simulink model "EV_Truck_Model"  (R2022b)
settings: Solver=FixedStepAuto  StartTime=0  StopTime=26553  FixedStep=0.1  RelTol=1e-3
model workspace (MAT data in the model file):
  ADAS_MaxAccel = 2
  ADAS_MaxDecel = 2.5
  Adas_on_off = 0
  Batt_cap_ah : Simulink.Parameter (value not decoded)
  Batt_rist_r0 : Simulink.Parameter (value not decoded)
  Batt_soc_s0 : Simulink.Parameter (value not decoded)
  Batt_volt_v0 : Simulink.Parameter (value not decoded)
  Motor_eff_100 : Simulink.Parameter (value not decoded)
  Motor_eff_190 : Simulink.Parameter (value not decoded)
  Motor_eff_95 : Simulink.Parameter (value not decoded)
  Motor_rpm_100 : Simulink.Parameter (value not decoded)
  Motor_rpm_190 : Simulink.Parameter (value not decoded)
  Motor_rpm_95 : Simulink.Parameter (value not decoded)
  Motor_torque_pos_100 : Simulink.Parameter (value not decoded)
  Motor_torque_pos_190 : Simulink.Parameter (value not decoded)
  Motor_torque_pos_95 : Simulink.Parameter (value not decoded)
  Motor_trq_190 : Simulink.Parameter (value not decoded)
  Motor_trq_95 : Simulink.Parameter (value not decoded)
  Sim_step = 0.1
  Test_DriveCycle = 0
  Trans_ratio = 6.142
  Veh_cog_fx = 1.69543
  Veh_cog_h = 0.605887
  Veh_cog_rx = 2.11956
  Veh_diff = 6.7
  Veh_whl_crr = 0.01
  Veh_whl_k = 180000
  Veh_whl_radius = 0.35
symbols that are objects in the model workspace (value not decoded): Motor_eff_100, Motor_eff_190, Motor_eff_95, Motor_rpm_100, Motor_rpm_190, Motor_rpm_95, Motor_torque_pos_100, Motor_torque_pos_190, Motor_torque_pos_95, Motor_trq_190, Motor_trq_95
undefined symbols (not defined in the file): Batt_soc_init, canChannel, Elec_aux_sw, Elec_rgn_sw, Power_option, speed, time, Veh_mass
libraries: batteryecm_lib x170, simulink x14, canmsglib x9, canlib x7, autolibshared x5, nesl_utility x4, fl_lib x3, drivingvehiclecontroller x3, hdlsllib x3, sim3dlib x1, sim3dautolib x1, vrlib x1
(part 6 of 11)

== system EV_Truck_Model/Accumulator System/Battery Pack/Simscape HV Battery/Battery Semi-Pack 1 ==
  Battery 7s6p1 : Subsystem
      settings: PortSchema="{\"entries\":[{\"content\":{\"sides\":[{\"content\":{\"connectorIds\":[]},\"type\":\"ConnectorPlacement.EquallySpacedRectSide\",\"uuid\":\"a0694fe7-d780-4483-a41f-a7ed21683973\"},{\"content\":{\"connectorIds\":[],\"side\":\"RIGHT\"},\"type\":\"ConnectorPlacement.EquallySpacedRectSide\",\"uuid\":\"39469ca5-beea-4553-8147-277bd4be0bbc\"},{\"content\":{\"connectorIds\":[\"LConn1\"],\"side\":\"TOP\"},\"type\":\"ConnectorPlacement.EquallySpacedRectSide\",\"uuid\":\"ededc17a-74df-4b2c-b94f-9a58df69fee7\"},{\"content\":{\"connectorIds\":[\"RConn1\"],\"side\":\"BOTTOM\"},\"type\":\"ConnectorPlacement.EquallySpacedRectSide\",\"uuid\":\"b7141beb-a775-4bdc-a667-5b3929cade8e\"}]},\"type\":\"ConnectorPlacement.EquallySpacedConnector\",\"uuid\":\"2df81f02-ea4e-4946-bfe6-2aa0de3e9d2a\"}],\"packageUris\":[\"http://schema.mathworks.com/mf0/Connector/R2020b\"],\"version\":\"1.0\"}"
  Battery 7s6p2 : Subsystem
      settings: PortSchema="{\"entries\":[{\"content\":{\"sides\":[{\"content\":{\"connectorIds\":[]},\"type\":\"ConnectorPlacement.EquallySpacedRectSide\",\"uuid\":\"a0694fe7-d780-4483-a41f-a7ed21683973\"},{\"content\":{\"connectorIds\":[],\"side\":\"RIGHT\"},\"type\":\"ConnectorPlacement.EquallySpacedRectSide\",\"uuid\":\"39469ca5-beea-4553-8147-277bd4be0bbc\"},{\"content\":{\"connectorIds\":[\"LConn1\"],\"side\":\"TOP\"},\"type\":\"ConnectorPlacement.EquallySpacedRectSide\",\"uuid\":\"ededc17a-74df-4b2c-b94f-9a58df69fee7\"},{\"content\":{\"connectorIds\":[\"RConn1\"],\"side\":\"BOTTOM\"},\"type\":\"ConnectorPlacement.EquallySpacedRectSide\",\"uuid\":\"b7141beb-a775-4bdc-a667-5b3929cade8e\"}]},\"type\":\"ConnectorPlacement.EquallySpacedConnector\",\"uuid\":\"2df81f02-ea4e-4946-bfe6-2aa0de3e9d2a\"}],\"packageUris\":[\"http://schema.mathworks.com/mf0/Connector/R2020b\"],\"version\":\"1.0\"}"
  Battery 7s6p3 : Subsystem
      settings: PortSchema="{\"entries\":[{\"content\":{\"sides\":[{\"content\":{\"connectorIds\":[]},\"type\":\"ConnectorPlacement.EquallySpacedRectSide\",\"uuid\":\"a0694fe7-d780-4483-a41f-a7ed21683973\"},{\"content\":{\"connectorIds\":[],\"side\":\"RIGHT\"},\"type\":\"ConnectorPlacement.EquallySpacedRectSide\",\"uuid\":\"39469ca5-beea-4553-8147-277bd4be0bbc\"},{\"content\":{\"connectorIds\":[\"LConn1\"],\"side\":\"TOP\"},\"type\":\"ConnectorPlacement.EquallySpacedRectSide\",\"uuid\":\"ededc17a-74df-4b2c-b94f-9a58df69fee7\"},{\"content\":{\"connectorIds\":[\"RConn1\"],\"side\":\"BOTTOM\"},\"type\":\"ConnectorPlacement.EquallySpacedRectSide\",\"uuid\":\"b7141beb-a775-4bdc-a667-5b3929cade8e\"}]},\"type\":\"ConnectorPlacement.EquallySpacedConnector\",\"uuid\":\"2df81f02-ea4e-4946-bfe6-2aa0de3e9d2a\"}],\"packageUris\":[\"http://schema.mathworks.com/mf0/Connector/R2020b\"],\"version\":\"1.0\"}"
  Battery 7s6p4 : Subsystem
      settings: PortSchema="{\"entries\":[{\"content\":{\"sides\":[{\"content\":{\"connectorIds\":[]},\"type\":\"ConnectorPlacement.EquallySpacedRectSide\",\"uuid\":\"a0694fe7-d780-4483-a41f-a7ed21683973\"},{\"content\":{\"connectorIds\":[],\"side\":\"RIGHT\"},\"type\":\"ConnectorPlacement.EquallySpacedRectSide\",\"uuid\":\"39469ca5-beea-4553-8147-277bd4be0bbc\"},{\"content\":{\"connectorIds\":[\"LConn1\"],\"side\":\"TOP\"},\"type\":\"ConnectorPlacement.EquallySpacedRectSide\",\"uuid\":\"ededc17a-74df-4b2c-b94f-9a58df69fee7\"},{\"content\":{\"connectorIds\":[\"RConn1\"],\"side\":\"BOTTOM\"},\"type\":\"ConnectorPlacement.EquallySpacedRectSide\",\"uuid\":\"b7141beb-a775-4bdc-a667-5b3929cade8e\"}]},\"type\":\"ConnectorPlacement.EquallySpacedConnector\",\"uuid\":\"2df81f02-ea4e-4946-bfe6-2aa0de3e9d2a\"}],\"packageUris\":[\"http://schema.mathworks.com/mf0/Connector/R2020b\"],\"version\":\"1.0\"}"
  Battery 7s6p5 : Subsystem
      settings: PortSchema="{\"entries\":[{\"content\":{\"sides\":[{\"content\":{\"connectorIds\":[]},\"type\":\"ConnectorPlacement.EquallySpacedRectSide\",\"uuid\":\"a0694fe7-d780-4483-a41f-a7ed21683973\"},{\"content\":{\"connectorIds\":[],\"side\":\"RIGHT\"},\"type\":\"ConnectorPlacement.EquallySpacedRectSide\",\"uuid\":\"39469ca5-beea-4553-8147-277bd4be0bbc\"},{\"content\":{\"connectorIds\":[\"LConn1\"],\"side\":\"TOP\"},\"type\":\"ConnectorPlacement.EquallySpacedRectSide\",\"uuid\":\"ededc17a-74df-4b2c-b94f-9a58df69fee7\"},{\"content\":{\"connectorIds\":[\"RConn1\"],\"side\":\"BOTTOM\"},\"type\":\"ConnectorPlacement.EquallySpacedRectSide\",\"uuid\":\"b7141beb-a775-4bdc-a667-5b3929cade8e\"}]},\"type\":\"ConnectorPlacement.EquallySpacedConnector\",\"uuid\":\"2df81f02-ea4e-4946-bfe6-2aa0de3e9d2a\"}],\"packageUris\":[\"http://schema.mathworks.com/mf0/Connector/R2020b\"],\"version\":\"1.0\"}"
  Battery 7s6p6 : Subsystem
      settings: PortSchema="{\"entries\":[{\"content\":{\"sides\":[{\"content\":{\"connectorIds\":[]},\"type\":\"ConnectorPlacement.EquallySpacedRectSide\",\"uuid\":\"a0694fe7-d780-4483-a41f-a7ed21683973\"},{\"content\":{\"connectorIds\":[],\"side\":\"RIGHT\"},\"type\":\"ConnectorPlacement.EquallySpacedRectSide\",\"uuid\":\"39469ca5-beea-4553-8147-277bd4be0bbc\"},{\"content\":{\"connectorIds\":[\"LConn1\"],\"side\":\"TOP\"},\"type\":\"ConnectorPlacement.EquallySpacedRectSide\",\"uuid\":\"ededc17a-74df-4b2c-b94f-9a58df69fee7\"},{\"content\":{\"connectorIds\":[\"RConn1\"],\"side\":\"BOTTOM\"},\"type\":\"ConnectorPlacement.EquallySpacedRectSide\",\"uuid\":\"b7141beb-a775-4bdc-a667-5b3929cade8e\"}]},\"type\":\"ConnectorPlacement.EquallySpacedConnector\",\"uuid\":\"2df81f02-ea4e-4946-bfe6-2aa0de3e9d2a\"}],\"packageUris\":[\"http://schema.mathworks.com/mf0/Connector/R2020b\"],\"version\":\"1.0\"}"
  High : PMIOPort  Side=Left
  Low : PMIOPort  Port=2  Side=Right
  connections:
  Battery 7s6p2/LConn1 -- Battery 7s6p1/RConn1
  High/RConn1 -- Battery 7s6p1/LConn1
  Battery 7s6p6/RConn1 -- Low/RConn1
  Battery 7s6p3/LConn1 -- Battery 7s6p2/RConn1
  Battery 7s6p4/LConn1 -- Battery 7s6p3/RConn1
  Battery 7s6p5/RConn1 -- Battery 7s6p6/LConn1
  Battery 7s6p5/LConn1 -- Battery 7s6p4/RConn1

== system EV_Truck_Model/Accumulator System/Battery Pack/Simscape HV Battery/Battery Semi-Pack 2 ==
  Battery 7s6p1 : Subsystem
      settings: PortSchema="{\"entries\":[{\"content\":{\"sides\":[{\"content\":{\"connectorIds\":[]},\"type\":\"ConnectorPlacement.EquallySpacedRectSide\",\"uuid\":\"a0694fe7-d780-4483-a41f-a7ed21683973\"},{\"content\":{\"connectorIds\":[],\"side\":\"RIGHT\"},\"type\":\"ConnectorPlacement.EquallySpacedRectSide\",\"uuid\":\"39469ca5-beea-4553-8147-277bd4be0bbc\"},{\"content\":{\"connectorIds\":[\"LConn1\"],\"side\":\"TOP\"},\"type\":\"ConnectorPlacement.EquallySpacedRectSide\",\"uuid\":\"ededc17a-74df-4b2c-b94f-9a58df69fee7\"},{\"content\":{\"connectorIds\":[\"RConn1\"],\"side\":\"BOTTOM\"},\"type\":\"ConnectorPlacement.EquallySpacedRectSide\",\"uuid\":\"b7141beb-a775-4bdc-a667-5b3929cade8e\"}]},\"type\":\"ConnectorPlacement.EquallySpacedConnector\",\"uuid\":\"2df81f02-ea4e-4946-bfe6-2aa0de3e9d2a\"}],\"packageUris\":[\"http://schema.mathworks.com/mf0/Connector/R2020b\"],\"version\":\"1.0\"}"
  Battery 7s6p2 : Subsystem
      settings: PortSchema="{\"entries\":[{\"content\":{\"sides\":[{\"content\":{\"connectorIds\":[]},\"type\":\"ConnectorPlacement.EquallySpacedRectSide\",\"uuid\":\"a0694fe7-d780-4483-a41f-a7ed21683973\"},{\"content\":{\"connectorIds\":[],\"side\":\"RIGHT\"},\"type\":\"ConnectorPlacement.EquallySpacedRectSide\",\"uuid\":\"39469ca5-beea-4553-8147-277bd4be0bbc\"},{\"content\":{\"connectorIds\":[\"LConn1\"],\"side\":\"TOP\"},\"type\":\"ConnectorPlacement.EquallySpacedRectSide\",\"uuid\":\"ededc17a-74df-4b2c-b94f-9a58df69fee7\"},{\"content\":{\"connectorIds\":[\"RConn1\"],\"side\":\"BOTTOM\"},\"type\":\"ConnectorPlacement.EquallySpacedRectSide\",\"uuid\":\"b7141beb-a775-4bdc-a667-5b3929cade8e\"}]},\"type\":\"ConnectorPlacement.EquallySpacedConnector\",\"uuid\":\"2df81f02-ea4e-4946-bfe6-2aa0de3e9d2a\"}],\"packageUris\":[\"http://schema.mathworks.com/mf0/Connector/R2020b\"],\"version\":\"1.0\"}"
  Battery 7s6p3 : Subsystem
      settings: PortSchema="{\"entries\":[{\"content\":{\"sides\":[{\"content\":{\"connectorIds\":[]},\"type\":\"ConnectorPlacement.EquallySpacedRectSide\",\"uuid\":\"a0694fe7-d780-4483-a41f-a7ed21683973\"},{\"content\":{\"connectorIds\":[],\"side\":\"RIGHT\"},\"type\":\"ConnectorPlacement.EquallySpacedRectSide\",\"uuid\":\"39469ca5-beea-4553-8147-277bd4be0bbc\"},{\"content\":{\"connectorIds\":[\"LConn1\"],\"side\":\"TOP\"},\"type\":\"ConnectorPlacement.EquallySpacedRectSide\",\"uuid\":\"ededc17a-74df-4b2c-b94f-9a58df69fee7\"},{\"content\":{\"connectorIds\":[\"RConn1\"],\"side\":\"BOTTOM\"},\"type\":\"ConnectorPlacement.EquallySpacedRectSide\",\"uuid\":\"b7141beb-a775-4bdc-a667-5b3929cade8e\"}]},\"type\":\"ConnectorPlacement.EquallySpacedConnector\",\"uuid\":\"2df81f02-ea4e-4946-bfe6-2aa0de3e9d2a\"}],\"packageUris\":[\"http://schema.mathworks.com/mf0/Connector/R2020b\"],\"version\":\"1.0\"}"
  Battery 7s6p4 : Subsystem
      settings: PortSchema="{\"entries\":[{\"content\":{\"sides\":[{\"content\":{\"connectorIds\":[]},\"type\":\"ConnectorPlacement.EquallySpacedRectSide\",\"uuid\":\"a0694fe7-d780-4483-a41f-a7ed21683973\"},{\"content\":{\"connectorIds\":[],\"side\":\"RIGHT\"},\"type\":\"ConnectorPlacement.EquallySpacedRectSide\",\"uuid\":\"39469ca5-beea-4553-8147-277bd4be0bbc\"},{\"content\":{\"connectorIds\":[\"LConn1\"],\"side\":\"TOP\"},\"type\":\"ConnectorPlacement.EquallySpacedRectSide\",\"uuid\":\"ededc17a-74df-4b2c-b94f-9a58df69fee7\"},{\"content\":{\"connectorIds\":[\"RConn1\"],\"side\":\"BOTTOM\"},\"type\":\"ConnectorPlacement.EquallySpacedRectSide\",\"uuid\":\"b7141beb-a775-4bdc-a667-5b3929cade8e\"}]},\"type\":\"ConnectorPlacement.EquallySpacedConnector\",\"uuid\":\"2df81f02-ea4e-4946-bfe6-2aa0de3e9d2a\"}],\"packageUris\":[\"http://schema.mathworks.com/mf0/Connector/R2020b\"],\"version\":\"1.0\"}"
  Battery 7s6p5 : Subsystem
      settings: PortSchema="{\"entries\":[{\"content\":{\"sides\":[{\"content\":{\"connectorIds\":[]},\"type\":\"ConnectorPlacement.EquallySpacedRectSide\",\"uuid\":\"a0694fe7-d780-4483-a41f-a7ed21683973\"},{\"content\":{\"connectorIds\":[],\"side\":\"RIGHT\"},\"type\":\"ConnectorPlacement.EquallySpacedRectSide\",\"uuid\":\"39469ca5-beea-4553-8147-277bd4be0bbc\"},{\"content\":{\"connectorIds\":[\"LConn1\"],\"side\":\"TOP\"},\"type\":\"ConnectorPlacement.EquallySpacedRectSide\",\"uuid\":\"ededc17a-74df-4b2c-b94f-9a58df69fee7\"},{\"content\":{\"connectorIds\":[\"RConn1\"],\"side\":\"BOTTOM\"},\"type\":\"ConnectorPlacement.EquallySpacedRectSide\",\"uuid\":\"b7141beb-a775-4bdc-a667-5b3929cade8e\"}]},\"type\":\"ConnectorPlacement.EquallySpacedConnector\",\"uuid\":\"2df81f02-ea4e-4946-bfe6-2aa0de3e9d2a\"}],\"packageUris\":[\"http://schema.mathworks.com/mf0/Connector/R2020b\"],\"version\":\"1.0\"}"
  Battery 7s6p6 : Subsystem
      settings: PortSchema="{\"entries\":[{\"content\":{\"sides\":[{\"content\":{\"connectorIds\":[]},\"type\":\"ConnectorPlacement.EquallySpacedRectSide\",\"uuid\":\"a0694fe7-d780-4483-a41f-a7ed21683973\"},{\"content\":{\"connectorIds\":[],\"side\":\"RIGHT\"},\"type\":\"ConnectorPlacement.EquallySpacedRectSide\",\"uuid\":\"39469ca5-beea-4553-8147-277bd4be0bbc\"},{\"content\":{\"connectorIds\":[\"LConn1\"],\"side\":\"TOP\"},\"type\":\"ConnectorPlacement.EquallySpacedRectSide\",\"uuid\":\"ededc17a-74df-4b2c-b94f-9a58df69fee7\"},{\"content\":{\"connectorIds\":[\"RConn1\"],\"side\":\"BOTTOM\"},\"type\":\"ConnectorPlacement.EquallySpacedRectSide\",\"uuid\":\"b7141beb-a775-4bdc-a667-5b3929cade8e\"}]},\"type\":\"ConnectorPlacement.EquallySpacedConnector\",\"uuid\":\"2df81f02-ea4e-4946-bfe6-2aa0de3e9d2a\"}],\"packageUris\":[\"http://schema.mathworks.com/mf0/Connector/R2020b\"],\"version\":\"1.0\"}"
  High : PMIOPort  Side=Left
  Low : PMIOPort  Port=2  Side=Right
  connections:
  Battery 7s6p2/LConn1 -- Battery 7s6p1/RConn1
  High/RConn1 -- Battery 7s6p1/LConn1
  Battery 7s6p6/RConn1 -- Low/RConn1
  Battery 7s6p3/LConn1 -- Battery 7s6p2/RConn1
  Battery 7s6p4/LConn1 -- Battery 7s6p3/RConn1
  Battery 7s6p5/RConn1 -- Battery 7s6p6/LConn1
  Battery 7s6p5/LConn1 -- Battery 7s6p4/RConn1

== system EV_Truck_Model/Accumulator System/Battery Pack/Simscape HV Battery/Battery Semi-Pack 3 ==
  Battery 7s6p1 : Subsystem
      settings: PortSchema="{\"entries\":[{\"content\":{\"sides\":[{\"content\":{\"connectorIds\":[]},\"type\":\"ConnectorPlacement.EquallySpacedRectSide\",\"uuid\":\"a0694fe7-d780-4483-a41f-a7ed21683973\"},{\"content\":{\"connectorIds\":[],\"side\":\"RIGHT\"},\"type\":\"ConnectorPlacement.EquallySpacedRectSide\",\"uuid\":\"39469ca5-beea-4553-8147-277bd4be0bbc\"},{\"content\":{\"connectorIds\":[\"LConn1\"],\"side\":\"TOP\"},\"type\":\"ConnectorPlacement.EquallySpacedRectSide\",\"uuid\":\"ededc17a-74df-4b2c-b94f-9a58df69fee7\"},{\"content\":{\"connectorIds\":[\"RConn1\"],\"side\":\"BOTTOM\"},\"type\":\"ConnectorPlacement.EquallySpacedRectSide\",\"uuid\":\"b7141beb-a775-4bdc-a667-5b3929cade8e\"}]},\"type\":\"ConnectorPlacement.EquallySpacedConnector\",\"uuid\":\"2df81f02-ea4e-4946-bfe6-2aa0de3e9d2a\"}],\"packageUris\":[\"http://schema.mathworks.com/mf0/Connector/R2020b\"],\"version\":\"1.0\"}"
  Battery 7s6p2 : Subsystem
      settings: PortSchema="{\"entries\":[{\"content\":{\"sides\":[{\"content\":{\"connectorIds\":[]},\"type\":\"ConnectorPlacement.EquallySpacedRectSide\",\"uuid\":\"a0694fe7-d780-4483-a41f-a7ed21683973\"},{\"content\":{\"connectorIds\":[],\"side\":\"RIGHT\"},\"type\":\"ConnectorPlacement.EquallySpacedRectSide\",\"uuid\":\"39469ca5-beea-4553-8147-277bd4be0bbc\"},{\"content\":{\"connectorIds\":[\"LConn1\"],\"side\":\"TOP\"},\"type\":\"ConnectorPlacement.EquallySpacedRectSide\",\"uuid\":\"ededc17a-74df-4b2c-b94f-9a58df69fee7\"},{\"content\":{\"connectorIds\":[\"RConn1\"],\"side\":\"BOTTOM\"},\"type\":\"ConnectorPlacement.EquallySpacedRectSide\",\"uuid\":\"b7141beb-a775-4bdc-a667-5b3929cade8e\"}]},\"type\":\"ConnectorPlacement.EquallySpacedConnector\",\"uuid\":\"2df81f02-ea4e-4946-bfe6-2aa0de3e9d2a\"}],\"packageUris\":[\"http://schema.mathworks.com/mf0/Connector/R2020b\"],\"version\":\"1.0\"}"
  Battery 7s6p3 : Subsystem
      settings: PortSchema="{\"entries\":[{\"content\":{\"sides\":[{\"content\":{\"connectorIds\":[]},\"type\":\"ConnectorPlacement.EquallySpacedRectSide\",\"uuid\":\"a0694fe7-d780-4483-a41f-a7ed21683973\"},{\"content\":{\"connectorIds\":[],\"side\":\"RIGHT\"},\"type\":\"ConnectorPlacement.EquallySpacedRectSide\",\"uuid\":\"39469ca5-beea-4553-8147-277bd4be0bbc\"},{\"content\":{\"connectorIds\":[\"LConn1\"],\"side\":\"TOP\"},\"type\":\"ConnectorPlacement.EquallySpacedRectSide\",\"uuid\":\"ededc17a-74df-4b2c-b94f-9a58df69fee7\"},{\"content\":{\"connectorIds\":[\"RConn1\"],\"side\":\"BOTTOM\"},\"type\":\"ConnectorPlacement.EquallySpacedRectSide\",\"uuid\":\"b7141beb-a775-4bdc-a667-5b3929cade8e\"}]},\"type\":\"ConnectorPlacement.EquallySpacedConnector\",\"uuid\":\"2df81f02-ea4e-4946-bfe6-2aa0de3e9d2a\"}],\"packageUris\":[\"http://schema.mathworks.com/mf0/Connector/R2020b\"],\"version\":\"1.0\"}"
  Battery 7s6p4 : Subsystem
      settings: PortSchema="{\"entries\":[{\"content\":{\"sides\":[{\"content\":{\"connectorIds\":[]},\"type\":\"ConnectorPlacement.EquallySpacedRectSide\",\"uuid\":\"a0694fe7-d780-4483-a41f-a7ed21683973\"},{\"content\":{\"connectorIds\":[],\"side\":\"RIGHT\"},\"type\":\"ConnectorPlacement.EquallySpacedRectSide\",\"uuid\":\"39469ca5-beea-4553-8147-277bd4be0bbc\"},{\"content\":{\"connectorIds\":[\"LConn1\"],\"side\":\"TOP\"},\"type\":\"ConnectorPlacement.EquallySpacedRectSide\",\"uuid\":\"ededc17a-74df-4b2c-b94f-9a58df69fee7\"},{\"content\":{\"connectorIds\":[\"RConn1\"],\"side\":\"BOTTOM\"},\"type\":\"ConnectorPlacement.EquallySpacedRectSide\",\"uuid\":\"b7141beb-a775-4bdc-a667-5b3929cade8e\"}]},\"type\":\"ConnectorPlacement.EquallySpacedConnector\",\"uuid\":\"2df81f02-ea4e-4946-bfe6-2aa0de3e9d2a\"}],\"packageUris\":[\"http://schema.mathworks.com/mf0/Connector/R2020b\"],\"version\":\"1.0\"}"
  Battery 7s6p5 : Subsystem
      settings: PortSchema="{\"entries\":[{\"content\":{\"sides\":[{\"content\":{\"connectorIds\":[]},\"type\":\"ConnectorPlacement.EquallySpacedRectSide\",\"uuid\":\"a0694fe7-d780-4483-a41f-a7ed21683973\"},{\"content\":{\"connectorIds\":[],\"side\":\"RIGHT\"},\"type\":\"ConnectorPlacement.EquallySpacedRectSide\",\"uuid\":\"39469ca5-beea-4553-8147-277bd4be0bbc\"},{\"content\":{\"connectorIds\":[\"LConn1\"],\"side\":\"TOP\"},\"type\":\"ConnectorPlacement.EquallySpacedRectSide\",\"uuid\":\"ededc17a-74df-4b2c-b94f-9a58df69fee7\"},{\"content\":{\"connectorIds\":[\"RConn1\"],\"side\":\"BOTTOM\"},\"type\":\"ConnectorPlacement.EquallySpacedRectSide\",\"uuid\":\"b7141beb-a775-4bdc-a667-5b3929cade8e\"}]},\"type\":\"ConnectorPlacement.EquallySpacedConnector\",\"uuid\":\"2df81f02-ea4e-4946-bfe6-2aa0de3e9d2a\"}],\"packageUris\":[\"http://schema.mathworks.com/mf0/Connector/R2020b\"],\"version\":\"1.0\"}"
  Battery 7s6p6 : Subsystem
      settings: PortSchema="{\"entries\":[{\"content\":{\"sides\":[{\"content\":{\"connectorIds\":[]},\"type\":\"ConnectorPlacement.EquallySpacedRectSide\",\"uuid\":\"a0694fe7-d780-4483-a41f-a7ed21683973\"},{\"content\":{\"connectorIds\":[],\"side\":\"RIGHT\"},\"type\":\"ConnectorPlacement.EquallySpacedRectSide\",\"uuid\":\"39469ca5-beea-4553-8147-277bd4be0bbc\"},{\"content\":{\"connectorIds\":[\"LConn1\"],\"side\":\"TOP\"},\"type\":\"ConnectorPlacement.EquallySpacedRectSide\",\"uuid\":\"ededc17a-74df-4b2c-b94f-9a58df69fee7\"},{\"content\":{\"connectorIds\":[\"RConn1\"],\"side\":\"BOTTOM\"},\"type\":\"ConnectorPlacement.EquallySpacedRectSide\",\"uuid\":\"b7141beb-a775-4bdc-a667-5b3929cade8e\"}]},\"type\":\"ConnectorPlacement.EquallySpacedConnector\",\"uuid\":\"2df81f02-ea4e-4946-bfe6-2aa0de3e9d2a\"}],\"packageUris\":[\"http://schema.mathworks.com/mf0/Connector/R2020b\"],\"version\":\"1.0\"}"
  High : PMIOPort  Side=Left
  Low : PMIOPort  Port=2  Side=Right
  connections:
  Battery 7s6p2/LConn1 -- Battery 7s6p1/RConn1
  High/RConn1 -- Battery 7s6p1/LConn1
  Battery 7s6p6/RConn1 -- Low/RConn1
  Battery 7s6p3/LConn1 -- Battery 7s6p2/RConn1
  Battery 7s6p4/LConn1 -- Battery 7s6p3/RConn1
  Battery 7s6p5/RConn1 -- Battery 7s6p6/LConn1
  Battery 7s6p5/LConn1 -- Battery 7s6p4/RConn1

== system EV_Truck_Model/Accumulator System/Battery Pack/Simscape HV Battery/Battery Semi-Pack 4 ==
  Battery 7s6p1 : Subsystem
      settings: PortSchema="{\"entries\":[{\"content\":{\"sides\":[{\"content\":{\"connectorIds\":[]},\"type\":\"ConnectorPlacement.EquallySpacedRectSide\",\"uuid\":\"a0694fe7-d780-4483-a41f-a7ed21683973\"},{\"content\":{\"connectorIds\":[],\"side\":\"RIGHT\"},\"type\":\"ConnectorPlacement.EquallySpacedRectSide\",\"uuid\":\"39469ca5-beea-4553-8147-277bd4be0bbc\"},{\"content\":{\"connectorIds\":[\"LConn1\"],\"side\":\"TOP\"},\"type\":\"ConnectorPlacement.EquallySpacedRectSide\",\"uuid\":\"ededc17a-74df-4b2c-b94f-9a58df69fee7\"},{\"content\":{\"connectorIds\":[\"RConn1\"],\"side\":\"BOTTOM\"},\"type\":\"ConnectorPlacement.EquallySpacedRectSide\",\"uuid\":\"b7141beb-a775-4bdc-a667-5b3929cade8e\"}]},\"type\":\"ConnectorPlacement.EquallySpacedConnector\",\"uuid\":\"2df81f02-ea4e-4946-bfe6-2aa0de3e9d2a\"}],\"packageUris\":[\"http://schema.mathworks.com/mf0/Connector/R2020b\"],\"version\":\"1.0\"}"
  Battery 7s6p2 : Subsystem
      settings: PortSchema="{\"entries\":[{\"content\":{\"sides\":[{\"content\":{\"connectorIds\":[]},\"type\":\"ConnectorPlacement.EquallySpacedRectSide\",\"uuid\":\"a0694fe7-d780-4483-a41f-a7ed21683973\"},{\"content\":{\"connectorIds\":[],\"side\":\"RIGHT\"},\"type\":\"ConnectorPlacement.EquallySpacedRectSide\",\"uuid\":\"39469ca5-beea-4553-8147-277bd4be0bbc\"},{\"content\":{\"connectorIds\":[\"LConn1\"],\"side\":\"TOP\"},\"type\":\"ConnectorPlacement.EquallySpacedRectSide\",\"uuid\":\"ededc17a-74df-4b2c-b94f-9a58df69fee7\"},{\"content\":{\"connectorIds\":[\"RConn1\"],\"side\":\"BOTTOM\"},\"type\":\"ConnectorPlacement.EquallySpacedRectSide\",\"uuid\":\"b7141beb-a775-4bdc-a667-5b3929cade8e\"}]},\"type\":\"ConnectorPlacement.EquallySpacedConnector\",\"uuid\":\"2df81f02-ea4e-4946-bfe6-2aa0de3e9d2a\"}],\"packageUris\":[\"http://schema.mathworks.com/mf0/Connector/R2020b\"],\"version\":\"1.0\"}"
  Battery 7s6p3 : Subsystem
      settings: PortSchema="{\"entries\":[{\"content\":{\"sides\":[{\"content\":{\"connectorIds\":[]},\"type\":\"ConnectorPlacement.EquallySpacedRectSide\",\"uuid\":\"a0694fe7-d780-4483-a41f-a7ed21683973\"},{\"content\":{\"connectorIds\":[],\"side\":\"RIGHT\"},\"type\":\"ConnectorPlacement.EquallySpacedRectSide\",\"uuid\":\"39469ca5-beea-4553-8147-277bd4be0bbc\"},{\"content\":{\"connectorIds\":[\"LConn1\"],\"side\":\"TOP\"},\"type\":\"ConnectorPlacement.EquallySpacedRectSide\",\"uuid\":\"ededc17a-74df-4b2c-b94f-9a58df69fee7\"},{\"content\":{\"connectorIds\":[\"RConn1\"],\"side\":\"BOTTOM\"},\"type\":\"ConnectorPlacement.EquallySpacedRectSide\",\"uuid\":\"b7141beb-a775-4bdc-a667-5b3929cade8e\"}]},\"type\":\"ConnectorPlacement.EquallySpacedConnector\",\"uuid\":\"2df81f02-ea4e-4946-bfe6-2aa0de3e9d2a\"}],\"packageUris\":[\"http://schema.mathworks.com/mf0/Connector/R2020b\"],\"version\":\"1.0\"}"
  Battery 7s6p4 : Subsystem
      settings: PortSchema="{\"entries\":[{\"content\":{\"sides\":[{\"content\":{\"connectorIds\":[]},\"type\":\"ConnectorPlacement.EquallySpacedRectSide\",\"uuid\":\"a0694fe7-d780-4483-a41f-a7ed21683973\"},{\"content\":{\"connectorIds\":[],\"side\":\"RIGHT\"},\"type\":\"ConnectorPlacement.EquallySpacedRectSide\",\"uuid\":\"39469ca5-beea-4553-8147-277bd4be0bbc\"},{\"content\":{\"connectorIds\":[\"LConn1\"],\"side\":\"TOP\"},\"type\":\"ConnectorPlacement.EquallySpacedRectSide\",\"uuid\":\"ededc17a-74df-4b2c-b94f-9a58df69fee7\"},{\"content\":{\"connectorIds\":[\"RConn1\"],\"side\":\"BOTTOM\"},\"type\":\"ConnectorPlacement.EquallySpacedRectSide\",\"uuid\":\"b7141beb-a775-4bdc-a667-5b3929cade8e\"}]},\"type\":\"ConnectorPlacement.EquallySpacedConnector\",\"uuid\":\"2df81f02-ea4e-4946-bfe6-2aa0de3e9d2a\"}],\"packageUris\":[\"http://schema.mathworks.com/mf0/Connector/R2020b\"],\"version\":\"1.0\"}"
  Battery 7s6p5 : Subsystem
      settings: PortSchema="{\"entries\":[{\"content\":{\"sides\":[{\"content\":{\"connectorIds\":[]},\"type\":\"ConnectorPlacement.EquallySpacedRectSide\",\"uuid\":\"a0694fe7-d780-4483-a41f-a7ed21683973\"},{\"content\":{\"connectorIds\":[],\"side\":\"RIGHT\"},\"type\":\"ConnectorPlacement.EquallySpacedRectSide\",\"uuid\":\"39469ca5-beea-4553-8147-277bd4be0bbc\"},{\"content\":{\"connectorIds\":[\"LConn1\"],\"side\":\"TOP\"},\"type\":\"ConnectorPlacement.EquallySpacedRectSide\",\"uuid\":\"ededc17a-74df-4b2c-b94f-9a58df69fee7\"},{\"content\":{\"connectorIds\":[\"RConn1\"],\"side\":\"BOTTOM\"},\"type\":\"ConnectorPlacement.EquallySpacedRectSide\",\"uuid\":\"b7141beb-a775-4bdc-a667-5b3929cade8e\"}]},\"type\":\"ConnectorPlacement.EquallySpacedConnector\",\"uuid\":\"2df81f02-ea4e-4946-bfe6-2aa0de3e9d2a\"}],\"packageUris\":[\"http://schema.mathworks.com/mf0/Connector/R2020b\"],\"version\":\"1.0\"}"
  Battery 7s6p6 : Subsystem
      settings: PortSchema="{\"entries\":[{\"content\":{\"sides\":[{\"content\":{\"connectorIds\":[]},\"type\":\"ConnectorPlacement.EquallySpacedRectSide\",\"uuid\":\"a0694fe7-d780-4483-a41f-a7ed21683973\"},{\"content\":{\"connectorIds\":[],\"side\":\"RIGHT\"},\"type\":\"ConnectorPlacement.EquallySpacedRectSide\",\"uuid\":\"39469ca5-beea-4553-8147-277bd4be0bbc\"},{\"content\":{\"connectorIds\":[\"LConn1\",\"LConn2\"],\"side\":\"TOP\"},\"type\":\"ConnectorPlacement.EquallySpacedRectSide\",\"uuid\":\"ededc17a-74df-4b2c-b94f-9a58df69fee7\"},{\"content\":{\"connectorIds\":[\"RConn1\"],\"side\":\"BOTTOM\"},\"type\":\"ConnectorPlacement.EquallySpacedRectSide\",\"uuid\":\"b7141beb-a775-4bdc-a667-5b3929cade8e\"}]},\"type\":\"ConnectorPlacement.EquallySpacedConnector\",\"uuid\":\"2df81f02-ea4e-4946-bfe6-2aa0de3e9d2a\"}],\"packageUris\":[\"http://schema.mathworks.com/mf0/Connector/R2020b\"],\"version\":\"1.0\"}"
  High : PMIOPort  Side=Left
  Low : PMIOPort  Port=2  Side=Right
  SOC : PMIOPort  Port=3  Side=Left
  connections:
  Battery 7s6p2/LConn1 -- Battery 7s6p1/RConn1
  High/RConn1 -- Battery 7s6p1/LConn1
  Battery 7s6p6/RConn1 -- Low/RConn1
  Battery 7s6p3/LConn1 -- Battery 7s6p2/RConn1
  Battery 7s6p4/LConn1 -- Battery 7s6p3/RConn1
  Battery 7s6p5/RConn1 -- Battery 7s6p6/LConn1
  Battery 7s6p5/LConn1 -- Battery 7s6p4/RConn1
  Battery 7s6p6/LConn2 -- SOC/RConn1

== system EV_Truck_Model/MCU and Motor System/Motor Torque Mapping and MCU Limiter/RPM Limiter/If Action Subsystem3 ==
  In1 : Inport
  Action Port : ActionPort  ActionPortLabel=if(u1 < 4500)
  Torque : Outport
  wires:
  In1/1 -> Torque/1

== system EV_Truck_Model/MCU and Motor System/Motor Torque Mapping and MCU Limiter/RPM Limiter/If Action Subsystem4 ==
  In1 : Inport
  Motor_RPM : Inport  Port=2
  Action Port : ActionPort  ActionPortLabel=elseif(u1 > 4500)
  Constant : Constant  Value=4600
  Constant1 : Constant  Value=100
  Divide : Product  Inputs=*/
  Minus : Sum  Inputs=+-
  Product : Product
  Torque : Outport
  wires:
  Product/1 -> Torque/1
  In1/1 -> Product/1
  Constant/1 -> Minus/1
  Motor_RPM/1 -> Minus/2
  Minus/1 -> Divide/1
  Constant1/1 -> Divide/2
  Divide/1 -> Product/2

== system EV_Truck_Model/MCU and Motor System/Motor Torque Mapping and MCU Limiter/Subsystem1/If Action Subsystem ==
  CurrentConsume : Inport
  Torque : Inport  Port=2
  Action Port : ActionPort  ActionPortLabel=elseif(u1 >= 350)
  Constant : Constant  Value=600
  Constant1 : Constant  Value=250
  Divide : Product  Inputs=*/
  Minus : Sum  Inputs=+-
  Product : Product
  Out1 : Outport
  wires:
  CurrentConsume/1 -> Minus/2
  Constant/1 -> Minus/1
  Minus/1 -> Divide/1
  Torque/1 -> Product/2
  Constant1/1 -> Divide/2
  Divide/1 -> Product/1
  Product/1 -> Out1/1

== system EV_Truck_Model/MCU and Motor System/Motor Torque Mapping and MCU Limiter/Subsystem1/If Action Subsystem1 ==
  Torque : Inport
  Action Port : ActionPort  ActionPortLabel=if(u1 < 350)
  Out1 : Outport
  wires:
  Torque/1 -> Out1/1

== system EV_Truck_Model/MCU and Motor System/Motor Torque Mapping and MCU Limiter/Torque Limit Map/100kW Motor ==
  RPM : Inport
  Action Port : ActionPort  ActionPortLabel=case [ 132 ]:
  1-D Lookup Table : Lookup_n-D  NumberOfTableDimensions=1  BreakpointsForDimension1=Motor_rpm_100  Table=Motor_torque_pos_100  InternalRulePriority=Speed  RndMeth=Simplest
  1-D Lookup TableNG : Lookup_n-D  NumberOfTableDimensions=1  BreakpointsForDimension1=Motor_rpm_100  Table=-0.8*Motor_torque_pos_100  InternalRulePriority=Speed  RndMeth=Simplest
  Out1 : Outport
  Out2 : Outport  Port=2
  wires:
  RPM/1 -> 1-D Lookup TableNG/1, 1-D Lookup Table/1
  1-D Lookup Table/1 -> Out1/1  "TrqLimit_max(Nm)"
  1-D Lookup TableNG/1 -> Out2/1  "TrqLimit_min(Nm)"

== system EV_Truck_Model/MCU and Motor System/Motor Torque Mapping and MCU Limiter/Torque Limit Map/190kW Motor ==
  RPM : Inport
  Action Port : ActionPort  ActionPortLabel=case [ 150 ]:
  1-D Lookup Table : Lookup_n-D  NumberOfTableDimensions=1  BreakpointsForDimension1=Motor_rpm_190  Table=Motor_torque_pos_190  InternalRulePriority=Speed  RndMeth=Simplest
  1-D Lookup TableNG : Lookup_n-D  NumberOfTableDimensions=1  BreakpointsForDimension1=Motor_rpm_190  Table=-0.8*Motor_torque_pos_190  InternalRulePriority=Speed  RndMeth=Simplest
  Out1 : Outport
  Out2 : Outport  Port=2
  wires:
  RPM/1 -> 1-D Lookup TableNG/1, 1-D Lookup Table/1
  1-D Lookup Table/1 -> Out1/1  "TrqLimit_max(Nm)"
  1-D Lookup TableNG/1 -> Out2/1  "TrqLimit_min(Nm)"

== system EV_Truck_Model/MCU and Motor System/Motor Torque Mapping and MCU Limiter/Torque Limit Map/95kW Motor ==
  RPM : Inport
  Action Port : ActionPort  ActionPortLabel=case [ 95 ]:
  1-D Lookup Table : Lookup_n-D  NumberOfTableDimensions=1  BreakpointsForDimension1=Motor_rpm_95  Table=Motor_torque_pos_95  InternalRulePriority=Speed  RndMeth=Simplest
  1-D Lookup TableNG : Lookup_n-D  NumberOfTableDimensions=1  BreakpointsForDimension1=Motor_rpm_95  Table=-0.8*Motor_torque_pos_95  InternalRulePriority=Speed  RndMeth=Simplest
  Out1 : Outport
  Out2 : Outport  Port=2
  wires:
  RPM/1 -> 1-D Lookup TableNG/1, 1-D Lookup Table/1
  1-D Lookup Table/1 -> Out1/1  "TrqLimit_max(Nm)"
  1-D Lookup TableNG/1 -> Out2/1  "TrqLimit_min(Nm)"

== system EV_Truck_Model/MCU and Motor System/Motor Torque Mapping and MCU Limiter/Torque Limiter/NormalTorque ==
  TrqCmd : Inport
  Action Port : ActionPort  ActionPortLabel=else
  Out1 : Outport
  wires:
  TrqCmd/1 -> Out1/1

== system EV_Truck_Model/MCU and Motor System/Motor Torque Mapping and MCU Limiter/Torque Limiter/Overtorque+ ==
  In1 : Inport
  Action Port : ActionPort  ActionPortLabel=if(u1 > u2)
  Out1 : Outport
  wires:
  In1/1 -> Out1/1

== system EV_Truck_Model/MCU and Motor System/Motor Torque Mapping and MCU Limiter/Torque Limiter/Overtorque- ==
  In1 : Inport
  Action Port : ActionPort  ActionPortLabel=elseif(u1 < u3)
  Out1 : Outport
  wires:
  In1/1 -> Out1/1

== system EV_Truck_Model/MCU and Motor System/Power and Efficiency Estimator/Auxiliary Power System/If Action Subsystem ==
  In1 : Inport
  Action Port : ActionPort  ActionPortLabel=if(u1 == 1)
  Add : Sum
  Idle Power : Constant  Value=1800
  Out1 : Outport
  wires:
  In1/1 -> Add/1
  Add/1 -> Out1/1
  Idle Power/1 -> Add/2

== system EV_Truck_Model/MCU and Motor System/Power and Efficiency Estimator/Auxiliary Power System/If Action Subsystem1 ==
  Action Port : ActionPort  ActionPortLabel=else
  Idle Power : Constant  Value=1800
  Out1 : Outport
  wires:
  Idle Power/1 -> Out1/1

== system EV_Truck_Model/MCU and Motor System/Power and Efficiency Estimator/Efficiency Map/100kW motor ==
  RPM : Inport
  TRQ POS : Inport  Port=2
  Action Port : ActionPort  ActionPortLabel=case [ 132 ]:
  2-D Lookup Table Eff 132kW : Lookup_n-D  BreakpointsForDimension1=[0:500:4500]  BreakpointsForDimension2=[0:100:1000]  Table=Motor_eff_100  InternalRulePriority=Speed  RndMeth=Simplest
      settings: InputPortMap=u0,u1
  Out1 : Outport
  wires:
  RPM/1 -> 2-D Lookup Table Eff 132kW/1
  TRQ POS/1 -> 2-D Lookup Table Eff 132kW/2
  2-D Lookup Table Eff 132kW/1 -> Out1/1  "Effeciency"

== system EV_Truck_Model/MCU and Motor System/Power and Efficiency Estimator/Efficiency Map/190kW motor ==
  RPM : Inport
  TRQ POS : Inport  Port=2
  Action Port : ActionPort  ActionPortLabel=case [ 150 ]:
  2-D Lookup Table Eff 190kW : Lookup_n-D  BreakpointsForDimension1=Motor_trq_190  BreakpointsForDimension2=Motor_rpm_190  Table=Motor_eff_190  InternalRulePriority=Speed  RndMeth=Simplest
      settings: InputPortMap=u0,u1
  Out1 : Outport
  wires:
  RPM/1 -> 2-D Lookup Table Eff 190kW/2
  TRQ POS/1 -> 2-D Lookup Table Eff 190kW/1
  2-D Lookup Table Eff 190kW/1 -> Out1/1  "Effeciency"

== system EV_Truck_Model/MCU and Motor System/Power and Efficiency Estimator/Efficiency Map/95kW motor ==
  RPM : Inport
  TRQ POS : Inport  Port=2
  Action Port : ActionPort  ActionPortLabel=case [ 95 ]:
  2-D Lookup Table Eff 95kW : Lookup_n-D  BreakpointsForDimension1=Motor_trq_95  BreakpointsForDimension2=Motor_rpm_95  Table=Motor_eff_95  InternalRulePriority=Speed  RndMeth=Simplest
      settings: InputPortMap=u0,u1
  Out1 : Outport
  wires:
  RPM/1 -> 2-D Lookup Table Eff 95kW/2
  TRQ POS/1 -> 2-D Lookup Table Eff 95kW/1
  2-D Lookup Table Eff 95kW/1 -> Out1/1  "Effeciency"

== system EV_Truck_Model/System I//O/Can Unpack A/Transformation/If Action Subsystem ==
  Action Port : ActionPort  ActionPortLabel=if(u1 == 4)
  Constant : Constant  Value=4
  Out1 : Outport
  wires:
  Constant/1 -> Out1/1

== system EV_Truck_Model/System I//O/Can Unpack A/Transformation/If Action Subsystem1 ==
  Action Port : ActionPort  ActionPortLabel=elseif(u1 == 5)
  Constant : Constant  Value=5
  Out1 : Outport
  wires:
  Constant/1 -> Out1/1

== system EV_Truck_Model/System I//O/Can Unpack A/Transformation/If Action Subsystem2 ==
  Action Port : ActionPort  ActionPortLabel=elseif(u1 == 6)
  Constant : Constant  Value=6
  Out1 : Outport
  wires:
  Constant/1 -> Out1/1

== system EV_Truck_Model/System I//O/Can Unpack A/Transformation/If Action Subsystem3 ==
  Action Port : ActionPort  ActionPortLabel=if(u1 == 0)
  Constant : Constant  Value=0
  Out1 : Outport
  wires:
  Constant/1 -> Out1/1

== system EV_Truck_Model/System I//O/Can Unpack A/Transformation/If Action Subsystem4 ==
  Action Port : ActionPort  ActionPortLabel=elseif(u1 == 1)
  Constant : Constant
  Out1 : Outport
  wires:
  Constant/1 -> Out1/1

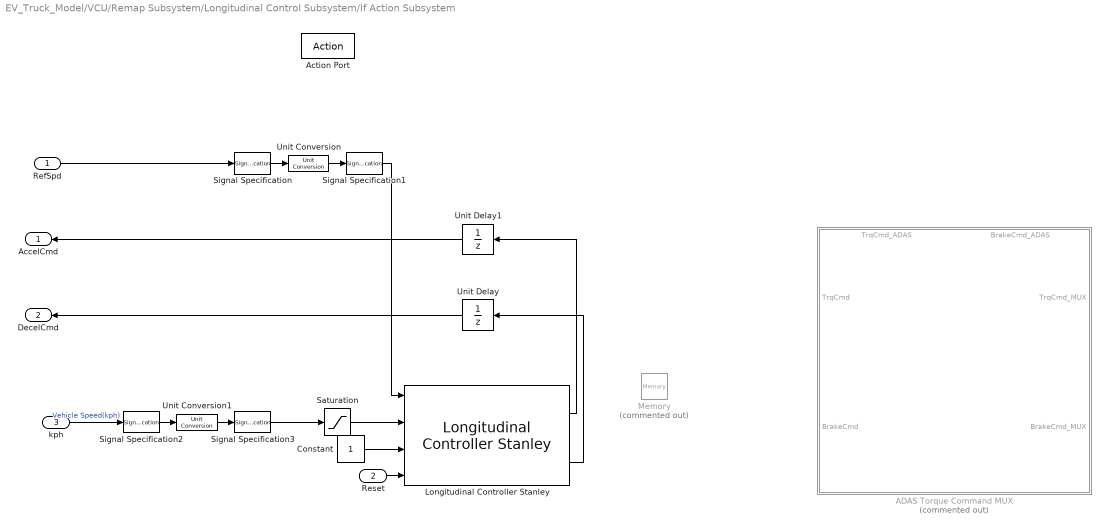
== system EV_Truck_Model/VCU/Remap Subsystem/Longitudinal Control Subsystem/If Action Subsystem ==
  RefSpd : Inport
  Reset : Inport  Port=2
  kph : Inport  Port=3
  Action Port : ActionPort  ActionPortLabel=if(u1 == 1)
  ADAS Torque Command MUX : Subsystem  Commented=on
      settings: PortSchema="{\"entries\":[{\"content\":{\"sides\":[{\"content\":{\"connectorIds\":[\"In1\",\"In2\"]},\"type\":\"ConnectorPlacement.EquallySpacedRectSide\",\"uuid\":\"6296c284-4aaa-4b65-bae8-92f6a1ca6334\"},{\"content\":{\"connectorIds\":[\"Out1\",\"Out2\"],\"side\":\"RIGHT\"},\"type\":\"ConnectorPlacement.EquallySpacedRectSide\",\"uuid\":\"12396655-9b4c-45e1-874c-981fa287baac\"},{\"content\":{\"connectorIds\":[\"In3\",\"In4\"],\"side\":\"TOP\"},\"type\":\"ConnectorPlacement.EquallySpacedRectSide\",\"uuid\":\"bc28bd2b-81fa-46c8-974f-c9b48ca64544\"}]},\"type\":\"ConnectorPlacement.EquallySpacedConnector\",\"uuid\":\"dc758841-edd4-411e-b954-73dcdfe0641a\"}],\"packageUris\":[\"http://schema.mathworks.com/mf0/Connector/R2020b\"],\"version\":\"1.0\"}"
  Constant : Constant
  Longitudinal Controller Stanley : drivingvehiclecontroller/Longitudinal Controller Stanley  Kp=2.5  Ki=1  SampleTime=Sim_step  MaxAcceleration=ADAS_MaxAccel  MaxDeceleration=ADAS_MaxDecel
  Memory : Memory  Commented=on
  Saturation : Saturate  UpperLimit=100  LowerLimit=0
  Signal Specification : SignalSpecification  Unit=km/hr
  Signal Specification1 : SignalSpecification  Unit=m/s
  Signal Specification2 : SignalSpecification  Unit=km/hr
  Signal Specification3 : SignalSpecification  Unit=m/s
  Unit Conversion : UnitConversion
  Unit Conversion1 : UnitConversion
  Unit Delay : UnitDelay  SampleTime=-1  HasFrameUpgradeWarning=on
  Unit Delay1 : UnitDelay  SampleTime=-1  HasFrameUpgradeWarning=on
  AccelCmd : Outport
  DecelCmd : Outport  Port=2
  wires:
  Signal Specification/1 -> Unit Conversion/1
  RefSpd/1 -> Signal Specification/1
  Longitudinal Controller Stanley/1 -> Unit Delay1/1
  Longitudinal Controller Stanley/2 -> Unit Delay/1
  kph/1 -> Signal Specification2/1  "Vehicle Speed(kph)"
  Unit Conversion1/1 -> Signal Specification3/1
  Unit Delay/1 -> DecelCmd/1
  Signal Specification3/1 -> Saturation/1
  Signal Specification2/1 -> Unit Conversion1/1
  Signal Specification1/1 -> Longitudinal Controller Stanley/1
  Reset/1 -> Longitudinal Controller Stanley/4
  Constant/1 -> Longitudinal Controller Stanley/3
  Unit Conversion/1 -> Signal Specification1/1
  Unit Delay1/1 -> AccelCmd/1
  Saturation/1 -> Longitudinal Controller Stanley/2

== system EV_Truck_Model/VCU/Remap Subsystem/Longitudinal Controller/ADAS Torque Command MUX ==
  TrqCmd : Inport
  BrakeCmd : Inport  Port=2
  TrqCmd_ADAS : Inport  Port=3
  BrakeCmd_ADAS : Inport  Port=4
  Constant : Constant  Value=0
  If : If  IfExpression=u1 == 1
  If Action Subsystem : Subsystem  TreatAsAtomicUnit=on
  If Action Subsystem1 : Subsystem  TreatAsAtomicUnit=on
  Merge : Merge
  Merge1 : Merge
  TrqCmd_MUX : Outport
  BrakeCmd_MUX : Outport  Port=2
  wires:
  TrqCmd/1 -> If Action Subsystem/1(TrqCmd)
  If Action Subsystem/1(Out1) -> Merge/1
  TrqCmd_ADAS/1 -> If Action Subsystem1/1(TrqCmd_ADAS)
  If Action Subsystem1/1(Out1) -> Merge/2
  Constant/1 -> If/1
  If/1 -> If Action Subsystem1/Action
  If/2 -> If Action Subsystem/Action
  Merge/1 -> TrqCmd_MUX/1
  BrakeCmd/1 -> If Action Subsystem/2(BrakeCmd)
  BrakeCmd_ADAS/1 -> If Action Subsystem1/2(BrakeCmd_ADAS)
  Merge1/1 -> BrakeCmd_MUX/1
  If Action Subsystem1/2(Out2) -> Merge1/2
  If Action Subsystem/2(Out2) -> Merge1/1

== system EV_Truck_Model/VCU/Remap Subsystem/TTC Calculator/Subsystem ==
  Dist : Inport
  In2 : Inport  Port=2
  Add : Sum  Inputs=+++++
  Multiply1 : Gain  Gain=1/5
  Subsystem : Subsystem
  Subsystem1 : Subsystem
  Subsystem2 : Subsystem
  Subsystem3 : Subsystem
  Subsystem4 : Subsystem
  Out1 : Outport
  wires:
  Subsystem1/1(Out1) -> Add/2
  Dist/1 -> Subsystem1/1(In1), Subsystem2/1(In1), Subsystem4/1(In1), Subsystem3/1(In1), Subsystem/1(In1)
  Subsystem/1(Out1) -> Add/1
  In2/1 -> Subsystem1/2(In2), Subsystem2/2(In2), Subsystem4/2(In2), Subsystem3/2(In2), Subsystem/2(In2)
  Subsystem3/1(Out1) -> Add/4
  Subsystem2/1(Out1) -> Add/3
  Add/1 -> Multiply1/1
  Subsystem4/1(Out1) -> Add/5
  Multiply1/1 -> Out1/1

== system EV_Truck_Model/Vehicle Dynamics System/Power Delivery and Braking System/BrakeSystem & Tyre Rolling Resistance/If Action Subsystem ==
  TyreForce_Fz(N) : Inport
  TyreForce_Rz(N) : Inport  Port=2
  Action Port : ActionPort  ActionPortLabel=if(u1 > 5)
  Multiply : Gain  Gain=Veh_whl_crr
  Multiply1 : Gain  Gain=Veh_whl_crr
  Out1 : Outport
  TyreForce_Resistance_Rx : Outport  Port=2
  wires:
  TyreForce_Rz(N)/1 -> Multiply1/1
  Multiply1/1 -> TyreForce_Resistance_Rx/1  "TyreForce_Resistance_Fx"
  Multiply/1 -> Out1/1  "TyreForce_Resistance_Fx"
  TyreForce_Fz(N)/1 -> Multiply/1

== system EV_Truck_Model/Vehicle Dynamics System/Power Delivery and Braking System/BrakeSystem & Tyre Rolling Resistance/If Action Subsystem1 ==
  TyreForce_Fz(N) : Inport
  TyreForce_Rz(N) : Inport  Port=2
  Vehicle_Speed(km/h) : Inport  Port=3
  Action Port : ActionPort  ActionPortLabel=else
  Multiply : Gain  Gain=Veh_whl_crr
  Multiply1 : Gain  Gain=Veh_whl_crr
  Multiply2 : Gain  Gain=1/5
  Product : Product
  Product1 : Product
  TyreForce_Resistance_Fx : Outport
  TyreForce_Resistance_Rx : Outport  Port=2
  wires:
  TyreForce_Rz(N)/1 -> Multiply1/1
  Product/1 -> TyreForce_Resistance_Rx/1  "TyreForce_Resistance_Rx"
  Multiply/1 -> Product1/1  "TyreForce_Resistance_Fx"
  TyreForce_Fz(N)/1 -> Multiply/1
  Vehicle_Speed(km/h)/1 -> Multiply2/1
  Multiply1/1 -> Product/1  "TyreForce_Resistance_Rx"
  Multiply2/1 -> Product1/2, Product/2
  Product1/1 -> TyreForce_Resistance_Fx/1  "TyreForce_Resistance_Rx"

== system EV_Truck_Model/Vehicle Dynamics System/Power Delivery and Braking System/BrakeSystem & Tyre Rolling Resistance/Subsystem ==
  note: Vehicle Stop olerance
  MotorSpeed : Inport
  BrakingForce : Inport  Port=2
  If : If  IfExpression=(-125 < u1) & (u1 < 125)  ElseIfExpressions=u1 > 0,u1 < 0  ShowElse=off
  If Action Subsystem : Subsystem  TreatAsAtomicUnit=on
  If Action Subsystem1 : Subsystem  TreatAsAtomicUnit=on
  If Action Subsystem2 : Subsystem  TreatAsAtomicUnit=on
  Merge : Merge  Inputs=3
  Multiply : Gain  Gain=0.6
  Multiply1 : Gain  Gain=0.4
  BFF : Outport
  BFR : Outport  Port=2
  wires:
  Multiply/1 -> BFF/1
  Multiply1/1 -> BFR/1
  MotorSpeed/1 -> If Action Subsystem/1(MotorSpeed), If/1
  BrakingForce/1 -> If Action Subsystem/2(BrakingForce), If Action Subsystem2/1(BrakingForce), If Action Subsystem1/1(BrakingForce)
  If/2 -> If Action Subsystem1/Action
  If Action Subsystem/1(Out1) -> Merge/1
  If Action Subsystem2/1(Out1) -> Merge/3
  Merge/1 -> Multiply1/1, Multiply/1
  If/1 -> If Action Subsystem/Action
  If/3 -> If Action Subsystem2/Action
  If Action Subsystem1/1(Out1) -> Merge/2

== system EV_Truck_Model/Accumulator System/Battery Pack/Simscape HV Battery/Battery Semi-Pack 1/Battery 7s6p1 ==
  Battery{1..7} (7 alike) : batteryecm_lib/Battery (Table-Based)  SOC_vec=Batt_soc_s0  T_dependence=simscape.enum.tablebattery.temperature_dependence.no  prm_dir=simscape.enum.tablebattery.prm_dir.noCurrentDirectionality  T_vec=[293] K  V0_mat=[2, 3, 3.2, 3.25, 3.25, 3.3, 3.3, 3.3, 3.35, 3.5] V  V0_vec=Batt_volt_v0 V  V_range=[0, inf] V  R0_mat=[15] mOhm  R0_vec=Batt_rist_r0 mOhm  R0_dis_mat=[.0117, .0085, .009; .011, .0085, .009; .0114, .0087, .0092; .0107, .0082, .0088; .0107, .0083, .0091; .0113, .0085, .0089; .0116, .0085, .0089] Ohm  R0_dis_vec=[.0085, .0085, .0087, .0082, .0083, .0085, .0085] Ohm  R0_ch_mat=[.0117, .0085, .009; .011, .0085, .009; .0114, .0087, .0092; .0107, .0082, .0088; .0107, .0083, .0091; .0113, .0085, .0089; .0116, .0085, .0089] Ohm  R0_ch_vec=[.0085, .0085, .0087, .0082, .0083, .0085, .0085] Ohm  AH=Batt_cap_ah A*hr  prm_leak=simscape.enum.tablebattery.prm_leak.disabled  Rleak_vec=[8000, 7000, 6000] Ohm  Rleak=7e3 Ohm  extrapolation_option=simscape.enum.extrapolation.nearest  SOC_port=simscape.enum.tablebattery.enable.no  prm_dyn=simscape.enum.tablebattery.prm_dyn.off  R1_mat=[.0109, .0029, .0013; .0069, .0024, .0012; .0047, .0026, .0013; .0034, .0016, .001; .0033, .0023, .0014; .0033, .0018, .0011; .0028, .0017, .0011] Ohm  R1_vec=[.0029, .0024, .0026, .0016, .0023, .0018, .0017] Ohm  tau1_mat=[20, 36, 39; 31, 45, 39; 109, 105, 61; 36, 29, 26; 59, 77, 67; 40, 33, 29; 25, 39, 33] s  tau1_vec=[36, 45, 105, 29, 77, 33, 39] s  R2_mat=[.0109, .0029, .0013; .0069, .0024, .0012; .0047, .0026, .0013; .0034, .0016, .001; .0033, .0023, .0014; .0033, .0018, .0011; .0028, .0017, .0011] Ohm  R2_vec=[.0029, .0024, .0026, .0016, .0023, .0018, .0017] Ohm  tau2_mat=[20, 36, 39; 31, 45, 39; 109, 105, 61; 36, 29, 26; 59, 77, 67; 40, 33, 29; 25, 39, 33] s  tau2_vec=[36, 45, 105, 29, 77, 33, 39] s  R3_mat=[.0109, .0029, .0013; .0069, .0024, .0012; .0047, .0026, .0013; .0034, .0016, .001; .0033, .0023, .0014; .0033, .0018, .0011; .0028, .0017, .0011] Ohm  R3_vec=[.0029, .0024, .0026, .0016, .0023, .0018, .0017] Ohm  tau3_mat=[20, 36, 39; 31, 45, 39; 109, 105, 61; 36, 29, 26; 59, 77, 67; 40, 33, 29; 25, 39, 33] s  tau3_vec=[36, 45, 105, 29, 77, 33, 39] s  R4_mat=[.0109, .0029, .0013; .0069, .0024, .0012; .0047, .0026, .0013; .0034, .0016, .001; .0033, .0023, .0014; .0033, .0018, .0011; .0028, .0017, .0011] Ohm  R4_vec=[.0029, .0024, .0026, .0016, .0023, .0018, .0017] Ohm  tau4_mat=[20, 36, 39; 31, 45, 39; 109, 105, 61; 36, 29, 26; 59, 77, 67; 40, 33, 29; 25, 39, 33] s  tau4_vec=[36, 45, 105, 29, 77, 33, 39] s  R5_mat=[.0109, .0029, .0013; .0069, .0024, .0012; .0047, .0026, .0013; .0034, .0016, .001; .0033, .0023, .0014; .0033, .0018, .0011; .0028, .0017, .0011] Ohm  R5_vec=[.0029, .0024, .0026, .0016, .0023, .0018, .0017] Ohm  tau5_mat=[20, 36, 39; 31, 45, 39; 109, 105, 61; 36, 29, 26; 59, 77, 67; 40, 33, 29; 25, 39, 33] s  tau5_vec=[36, 45, 105, 29, 77, 33, 39] s  prm_fade=simscape.enum.tablebattery.prm_fade.disabled  N0=100  dV0=0  dR0=0  dAH=0  dRleak=0  dR1=0  dR2=0  dR3=0  dR4=0  dR5=0  N0vec=[100, 200, 300]  Tfadevec=[298.15, 323.15] K  dV0vec=[0, 0, 0]  dR0vec=[0, 0, 0]  dAHvec=[0, 0, 0]  dRleakvec=[0, 0, 0]  dR1vec=[0, 0, 0]  dR2vec=[0, 0, 0]  dR3vec=[0, 0, 0]  dR4vec=[0, 0, 0]  dR5vec=[0, 0, 0]  dV0mat=[0, 0; 0, 0; 0, 0]  dR0mat=[0, 0; 0, 0; 0, 0]  dAHmat=[0, 0; 0, 0; 0, 0]  dRleakmat=[0, 0; 0, 0; 0, 0]  dR1mat=[0, 0; 0, 0; 0, 0]  dR2mat=[0, 0; 0, 0; 0, 0]  dR3mat=[0, 0; 0, 0; 0, 0]  dR4mat=[0, 0; 0, 0; 0, 0]  dR5mat=[0, 0; 0, 0; 0, 0]  prm_age_modeling=simscape.enum.tablebattery.prm_age_modeling.equation  storage_dt_age_vec=[0] d  storage_T_age_vec=[273] K  prm_age_OCV=simscape.enum.tablebattery.prm_age_OCV.OCV  OCV_age=0.9  SOC_age=0.6  prm_age_resistance=simscape.enum.tablebattery.prm_age.disabled  OCV_scaling_age_resistance=2.2134e6  OCV_offset_age_resistance=1.632e6  temp_exp_age_resistance=0.515833569 V  t_exp_age_resistance=0.75  T_age_vec_resistance=[273.15, 298.15, 323.15] K  dt_age_vec_resistance=[90, 180, 270, 360] d  dR0_age_vec=[0, 0, 0]  t_meas_dR0_age=100 d  dR0_age_mat=[0, 0, 0; 0, 0, 0; 0, 0, 0; 0, 0, 0]  prm_age_capacity=simscape.enum.tablebattery.prm_age.disabled  OCV_scaling_age_capacity=1.5097e07  OCV_offset_age_capacity=8.3625e06  temp_exp_age_capacity=0.6011 V  t_exp_age_capacity=0.75  T_age_vec_capacity=[273.15, 298.15, 323.15] K  dt_age_vec_capacity=[90, 180, 270, 360] d  dAH_age_vec=[0, 0, 0]  t_meas_dAH_age=100 d  dAH_age_mat=[0, 0, 0; 0, 0, 0; 0, 0, 0; 0, 0, 0]  thermal_port=simscape.enum.thermaleffects.omit  temperature=298.15 K  thermal_mass=100 J/K  i_specify=off  i_priority=None  i=0 A  i_nominal_specify=off  i_nominal_unit=A  i_nominal_value=1  v_specify=off  v_priority=None  v=0 V  v_nominal_specify=off  v_nominal_unit=V  v_nominal_value=1  stateOfCharge_specify=on  stateOfCharge_priority=High  stateOfCharge=Batt_soc_init  stateOfCharge_nominal_specify=off  stateOfCharge_nominal_unit=1  stateOfCharge_nominal_value=1  num_cycles_specify=off  num_cycles_priority=High  num_cycles=0  num_cycles_nominal_specify=off  num_cycles_nominal_unit=1  num_cycles_nominal_value=1  cell_temperature_specify=off  cell_temperature_priority=High  cell_temperature=298.15 K  cell_temperature_nominal_specify=off  cell_temperature_nominal_unit=K  cell_temperature_nominal_value=1
      settings: InternalSimscapePortConfiguration="{\"Bottom\":[],\"Left\":[{\"id\":\"p\",\"label\":\"+\",\"type\":\"foundation.electrical.electrical\"}],\"Right\":[{\"id\":\"n\",\"label\":\"-\",\"type\":\"foundation.electrical.electrical\"}],\"Top\":[]}"
  High : PMIOPort  Side=Left
  Low : PMIOPort  Port=2  Side=Right
  connections:
  Low/RConn1 -- Battery7/RConn1
  Battery1/LConn1 -- High/RConn1
  Battery2/LConn1 -- Battery1/RConn1
  Battery3/LConn1 -- Battery2/RConn1
  Battery4/LConn1 -- Battery3/RConn1
  Battery5/LConn1 -- Battery4/RConn1
  Battery6/LConn1 -- Battery5/RConn1
  Battery7/LConn1 -- Battery6/RConn1
